simulink model "first_tap_test"  (Simulink 7.2)
settings: Solver=VariableStepDiscrete  StartTime=0.0  StopTime=50  RelTol=1e-3
undefined symbols (not defined in the file or in its folder): pfb_coeff_gen_calc
libraries: xbsIndex_r4 x45, casper_library_misc x3, casper_library_delays x2, simulink x1
settings Model: Creator=User  LastModifiedBy=root
settings OptimizationCC: InitFltsAndDblsToZero=on
settings DebuggingCC: SaveWithDisabledLinksMsg=none  SaveWithParameterizedLinksMsg=none

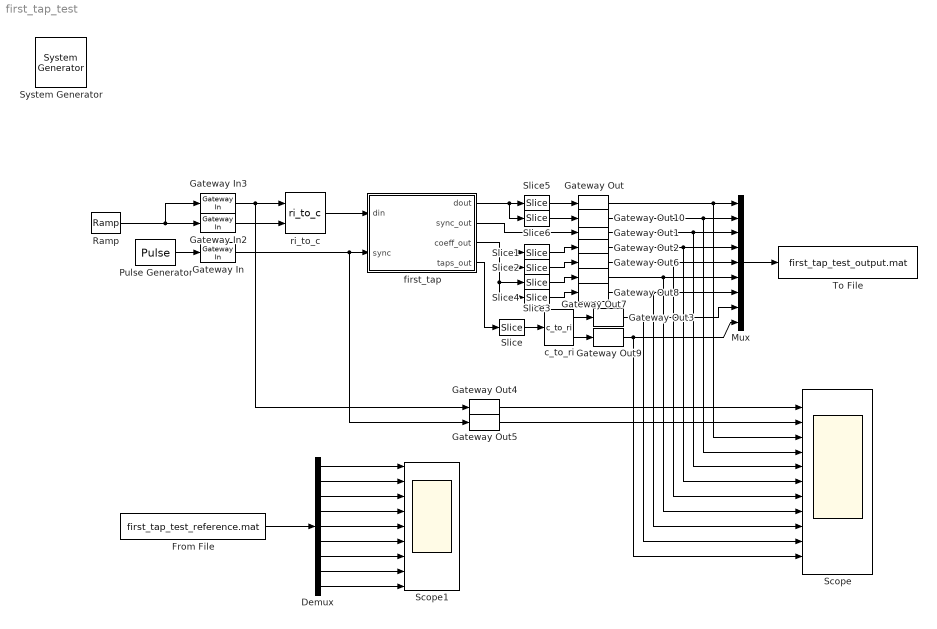
== system first_tap_test ==
  " System Generator" : xbsIndex_r4/ System Generator  Tag=genX  SystemSampleTime=-1  xilinxfamily=Virtex4  part=xc4vsx35  speed=-10  package=ff668  synthesis_tool=XST  clock_wrapper=Clock Enables  directory=./netlist  testbench=off  simulink_period=1  sysclk_period=100  dcm_input_clock_period=100  incr_netlist=off  trim_vbits=Everywhere in SubSystem  dbl_ovrd=According to Block Masks  core_generation=According to Block Masks  run_coregen=off  deprecated_control=off  eval_field=0  block_type=sysgen
      settings: block_version=10.1.1
  Demux : Demux  Outputs=9
  From File : FromFile  FileName=first_tap_test_reference.mat  SampleTime=1
  Gateway In : xbsIndex_r4/Gateway In  arith_type=Boolean  n_bits=16  bin_pt=14  quantization="Round  (unbiased: +/- Inf)"  overflow=Saturate  period=1  dbl_ovrd=off  timing_constraint=None  locs_specified=off  LOCs={}  hdl_port=on  block_type=gatewayin
      settings: infoedit="Gateway in block.  Converts inputs of type Simulink integer, double and fixed point to  Xilinx fixed point type.<P><P>Hardware notes:  In hardware these blocks become top level input ports."  block_version=10.1.1
  Gateway In2 : xbsIndex_r4/Gateway In  arith_type="Signed  (2's comp)"  n_bits=8  bin_pt=7  quantization=Truncate  overflow=Wrap  period=1  dbl_ovrd=off  timing_constraint=None  locs_specified=off  LOCs={}  hdl_port=on  block_type=gatewayin
      settings: infoedit="Gateway in block.  Converts inputs of type Simulink integer, double and fixed point to  Xilinx fixed point type.<P><P>Hardware notes:  In hardware these blocks become top level input ports."  block_version=10.1.1
  Gateway In3 : xbsIndex_r4/Gateway In  arith_type="Signed  (2's comp)"  n_bits=8  bin_pt=7  quantization=Truncate  overflow=Wrap  period=1  dbl_ovrd=off  timing_constraint=None  locs_specified=off  LOCs={}  hdl_port=on  block_type=gatewayin
      settings: infoedit="Gateway in block.  Converts inputs of type Simulink integer, double and fixed point to  Xilinx fixed point type.<P><P>Hardware notes:  In hardware these blocks become top level input ports."  block_version=10.1.1
  Gateway Out{,1..10} (11 alike) : xbsIndex_r4/Gateway Out  hdl_port=on  timing_constraint=None  locs_specified=off  LOCs={}  block_type=gatewayout
      settings: infoedit="Gateway out block.  Converts Xilinx fixed point inputs into ouputs of type Simulink integer, double, or fixed point.<P><P>Hardware notes:  In hardware these blocks become top level output ports or are discarded, depending on how they are configured."  block_version=10.1.1
  Mux : Mux  Inputs=9
  Pulse Generator : DiscretePulseGenerator  Period=16  PhaseDelay=7
  Ramp : simulink/Sources/Ramp  SystemSampleTime=-1  slope=1/64  start=0  X0=0
  Scope : Scope  NumInputPorts=11
      settings: YMin=-1~-1~-1~-5~-5~-5~-5~-5~-5~-5~-5  YMax=1~2~1~5~5~5~5~5~5~5~5
  Scope1 : Scope  NumInputPorts=9
      settings: YMin=-5~-5~-5~-5~-5~-5~-5~-5~-5  YMax=5~5~5~5~5~5~5~5~5
  Slice : xbsIndex_r4/Slice  nbits=28  boolean_output=off  mode=Upper Bit Location + Width  bit1=0  base1=MSB of Input  bit0=0  base0=LSB of Input  dbl_ovrd=off  block_type=slice
      settings: infoedit="Extracts a given range of bits from each input sample and presents it at the output.  The output type is ordinarily unsigned with binary point at zero, but can be Boolean when the slice is one bit wide.<P><P>Hardware notes: In hardware this block costs nothing."  block_version=10.1.1
  Slice1 : xbsIndex_r4/Slice  nbits=6  boolean_output=off  mode=Two Bit Locations  bit1=0  base1=MSB of Input  bit0=-5  base0=MSB of Input  dbl_ovrd=off  block_type=slice
      settings: infoedit="Extracts a given range of bits from each input sample and presents it at the output.  The output type is ordinarily unsigned with binary point at zero, but can be Boolean when the slice is one bit wide.<P><P>Hardware notes: In hardware this block costs nothing."  block_version=10.1.1
  Slice2 : xbsIndex_r4/Slice  nbits=6  boolean_output=off  mode=Two Bit Locations  bit1=-6  base1=MSB of Input  bit0=-11  base0=MSB of Input  dbl_ovrd=off  block_type=slice
      settings: infoedit="Extracts a given range of bits from each input sample and presents it at the output.  The output type is ordinarily unsigned with binary point at zero, but can be Boolean when the slice is one bit wide.<P><P>Hardware notes: In hardware this block costs nothing."  block_version=10.1.1
  Slice3 : xbsIndex_r4/Slice  nbits=6  boolean_output=off  mode=Two Bit Locations  bit1=-12  base1=MSB of Input  bit0=-17  base0=MSB of Input  dbl_ovrd=off  block_type=slice
      settings: infoedit="Extracts a given range of bits from each input sample and presents it at the output.  The output type is ordinarily unsigned with binary point at zero, but can be Boolean when the slice is one bit wide.<P><P>Hardware notes: In hardware this block costs nothing."  block_version=10.1.1
  Slice4 : xbsIndex_r4/Slice  nbits=6  boolean_output=off  mode=Two Bit Locations  bit1=-18  base1=MSB of Input  bit0=-23  base0=MSB of Input  dbl_ovrd=off  block_type=slice
      settings: infoedit="Extracts a given range of bits from each input sample and presents it at the output.  The output type is ordinarily unsigned with binary point at zero, but can be Boolean when the slice is one bit wide.<P><P>Hardware notes: In hardware this block costs nothing."  block_version=10.1.1
  Slice5 : xbsIndex_r4/Slice  nbits=6  boolean_output=off  mode=Two Bit Locations  bit1=0  base1=MSB of Input  bit0=-7  base0=MSB of Input  dbl_ovrd=off  block_type=slice
      settings: infoedit="Extracts a given range of bits from each input sample and presents it at the output.  The output type is ordinarily unsigned with binary point at zero, but can be Boolean when the slice is one bit wide.<P><P>Hardware notes: In hardware this block costs nothing."  block_version=10.1.1
  Slice6 : xbsIndex_r4/Slice  nbits=6  boolean_output=off  mode=Two Bit Locations  bit1=0  base1=MSB of Input  bit0=-7  base0=MSB of Input  dbl_ovrd=off  block_type=slice
      settings: infoedit="Extracts a given range of bits from each input sample and presents it at the output.  The output type is ordinarily unsigned with binary point at zero, but can be Boolean when the slice is one bit wide.<P><P>Hardware notes: In hardware this block costs nothing."  block_version=10.1.1
  To File : ToFile  Filename=first_tap_test_output.mat  MatrixName=output
  c_to_ri : casper_library_misc/c_to_ri  SystemSampleTime=-1  n_bits=14  bin_pt=12
      settings: AttributesFormatString=14_12 r/i
  first_tap : Subsystem  AncestorBlock=casper_library_pfbs/first_tap  mask(first_tap){nput=0, PFBSize=5, CoeffBitWidth=6, TotalTaps=5, BitWidthIn=8, CoeffDistMem=1, WindowType=bartlett, mult_latency=3, bram_latency=2, n_inputs=1, fwidth=1, use_hdl=off, use_embedded=off}
      mask prompts: nput "This is input number:"; PFBSize "Size of PFB: (2^? pnts)"; CoeffBitWidth "Bitwidth of Coefficients:"; TotalTaps "Total Number of Taps:"; BitWidthIn "Input Bitwidth:"; CoeffDistMem "Implement Coeff Gen in Distributed Memory:"; WindowType "Windowing Function:"; mult_latency "Mult Latency"; bram_latency "BRAM Latency"; n_inputs "Number of Simultaneous Inputs: (2^?)"; fwidth "Bit Width (normal=1)"; use_hdl "Use behavioral HDL for multlipliers"; use_embedded "Use embedded multipliers"
      mask init:
      | first_tap_init(gcb,...
      |     'nput', nput,...
      |     'PFBSize', PFBSize,...
      |     'CoeffBitWidth', CoeffBitWidth,...
      |     'TotalTaps', TotalTaps,...
      |     'BitWidthIn', BitWidthIn,...
      |     'CoeffDistMem', CoeffDistMem,...
      |     'WindowType', WindowType,...
      |     'mult_latency', mult_latency,...
      |     'bram_latency', bram_latency,...
      |     'n_inputs', n_inputs,...
      |     'fwidth', fwidth,...
      |     'use_hdl', use_hdl,...
      |     'use_embedded', use_embedded);
      settings: AttributesFormatString=input=0, taps=5
      mask StyleString: edit,edit,edit,edit,edit,edit,popup(bartlett|barthannwin|blackman|blackmanharris|bohamwin|chebwin|flattopwin|gausswin|hamming|hann|kaiser|nuttallwin|parzenwin|rectwin|tukeywin|triang),edit,edit,edit,edit,checkbox,checkbox
      mask CallbackString:
      | |||||||||||use_hdl = get_param(gcb,'use_hdl');
      | if( strcmp(use_hdl,'on')),
      |     set_param(gcb, 'use_embedded','off');
      |     set_param(gcb, 'MaskVisibilities',{'on','on','on','on','on','on','on','on','on','on','on','on','off'});
      | else,
      |     set_param(gcb, 'MaskVisibilities',{'on','on','on','on','on','on','on','on','on','on','on','on','on'});
      | end
      | |
  ri_to_c : casper_library_misc/ri_to_c  SystemSampleTime=-1
  wires:
  Pulse Generator/1 -> Gateway In/1
  Gateway In/1 -> Gateway Out5/1, first_tap/2(sync)
  Ramp/1 -> Gateway In2/1, Gateway In3/1
  c_to_ri/1 -> Gateway Out3/1
  Gateway Out4/1 -> Scope/1
  Gateway Out5/1 -> Scope/2
  Gateway Out/1 -> Scope/3, Mux/1
  Gateway Out3/1 -> Scope/10, Mux/8
  Gateway In3/1 -> Gateway Out4/1, ri_to_c/1
  Gateway In2/1 -> ri_to_c/2
  c_to_ri/2 -> Gateway Out9/1
  Gateway Out9/1 -> Scope/11, Mux/9
  Slice/1 -> c_to_ri/1
  ri_to_c/1 -> first_tap/1(din)
  first_tap/1(dout) -> Slice5/1, Slice6/1
  first_tap/2(sync_out) -> Gateway Out1/1
  first_tap/4(taps_out) -> Slice/1
  first_tap/3(coeff_out) -> Slice1/1, Slice2/1, Slice3/1, Slice4/1
  Slice1/1 -> Gateway Out2/1
  Slice2/1 -> Gateway Out6/1
  Slice3/1 -> Gateway Out7/1
  Slice4/1 -> Gateway Out8/1
  Slice5/1 -> Gateway Out/1
  Slice6/1 -> Gateway Out10/1
  Gateway Out10/1 -> Scope/4, Mux/2
  Gateway Out1/1 -> Scope/5, Mux/3
  Gateway Out2/1 -> Scope/6, Mux/4
  Gateway Out6/1 -> Scope/7, Mux/5
  Gateway Out7/1 -> Scope/8, Mux/6
  Gateway Out8/1 -> Scope/9, Mux/7
  Mux/1 -> To File/1
  From File/1 -> Demux/1
  Demux/1 -> Scope1/1
  Demux/2 -> Scope1/2
  Demux/3 -> Scope1/3
  Demux/4 -> Scope1/4
  Demux/5 -> Scope1/5
  Demux/6 -> Scope1/6
  Demux/7 -> Scope1/7
  Demux/8 -> Scope1/8
  Demux/9 -> Scope1/9

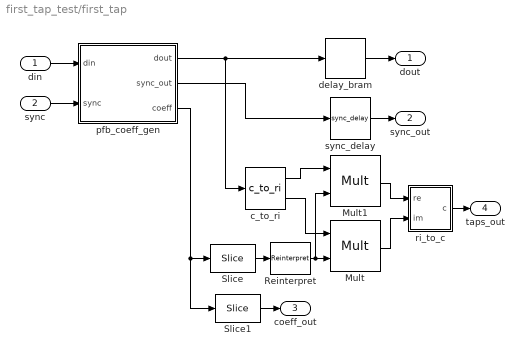
== system first_tap_test/first_tap ==
  din : Inport  OutDataType=sfix(16)  OutScaling=2^0
  sync : Inport  Port=2  OutDataType=sfix(16)  OutScaling=2^0
  Mult : xbsIndex_r4/Mult  precision=Full  arith_type="Signed  (2's comp)"  n_bits=8  bin_pt=2  quantization=Truncate  overflow=Wrap  en=off  latency=mult_latency  dbl_ovrd=off  use_behavioral_HDL=off  opt=Speed  use_embedded=off  optimum_pipeline=off  pipeline=on  use_rpm=on  placement_style=Rectangular shape  block_type=mult
      settings: infoedit=Hardware notes: To use the internal pipeline stage of the dedicated multiplier you must select 'Pipeline for maximum performance'.  xl_area=[0, 0, 0, 0, 0, 0, 0]  block_version=9.1.01
  Mult1 : xbsIndex_r4/Mult  precision=Full  arith_type="Signed  (2's comp)"  n_bits=8  bin_pt=2  quantization=Truncate  overflow=Wrap  en=off  latency=mult_latency  dbl_ovrd=off  use_behavioral_HDL=off  opt=Speed  use_embedded=off  optimum_pipeline=off  pipeline=on  use_rpm=on  placement_style=Rectangular shape  block_type=mult
      settings: infoedit=Hardware notes: To use the internal pipeline stage of the dedicated multiplier you must select 'Pipeline for maximum performance'.  xl_area=[0, 0, 0, 0, 0, 0, 0]  block_version=9.1.01
  Reinterpret : xbsIndex_r4/Reinterpret  force_arith_type=on  arith_type="Signed  (2's comp)"  force_bin_pt=on  bin_pt=CoeffBitWidth - 1  block_type=reinterpret
      settings: infoedit="Changes signal type without altering the binary representation.   You can changed the signal between signed and unsigned, and relocate the binary point.<P><P>Hardware notes: In hardware this block costs nothing.<P><P>Example:  Suppose the input is 6 bits wide, signed, with 2 fractional bits, and the output is forced to unsigned with 0 fractional bits.  Then an input of -2.0 (1110.00 in binary 2's complement) becomes an output of 56 (111000 in binary)."  block_version=9.1.01
  Slice : xbsIndex_r4/Slice  nbits=CoeffBitWidth  boolean_output=off  mode=Lower Bit Location + Width  bit1=0  base1=MSB of Input  bit0=0  base0=LSB of Input  dbl_ovrd=off  block_type=slice
      settings: infoedit="Extracts a given range of bits from each input sample and presents it at the output.  The output type is ordinarily unsigned with binary point at zero, but can be Boolean when the slice is one bit wide.<P><P>Hardware notes: In hardware this block costs nothing."  block_version=9.1.01
  Slice1 : xbsIndex_r4/Slice  nbits=CoeffBitWidth * (TotalTaps - 1)  boolean_output=off  mode=Two Bit Locations  bit1=0  base1=MSB of Input  bit0=CoeffBitWidth  base0=LSB of Input  dbl_ovrd=off  block_type=slice
      settings: infoedit="Extracts a given range of bits from each input sample and presents it at the output.  The output type is ordinarily unsigned with binary point at zero, but can be Boolean when the slice is one bit wide.<P><P>Hardware notes: In hardware this block costs nothing."  block_version=9.1.01
  c_to_ri : casper_library_misc/c_to_ri  SystemSampleTime=-1  n_bits=BitWidthIn  bin_pt=BitWidthIn-1
      settings: AttributesFormatString=8_7 r/i
  delay_bram : casper_library_delays/delay_bram  SystemSampleTime=-1  DelayLen=2^(PFBSize-n_inputs)  bram_latency=bram_latency
  pfb_coeff_gen : Subsystem  AncestorBlock=casper_library_pfbs/pfb_coeff_gen  mask(pfb_coeff_gen){PFBSize=5, CoeffBitWidth=6, TotalTaps=5, CoeffDistMem=1, WindowType=bartlett, bram_latency=2, n_inputs=1, nput=0, fwidth=1}
      mask prompts: PFBSize "Size of PFB: (2^? pnts)"; CoeffBitWidth "Bitwidth of Coefficients:"; TotalTaps "Total Number of Taps:"; CoeffDistMem "Implement Coeff Gen in Distributed Memory"; WindowType "Windowing Function:"; bram_latency "BRAM Latency"; n_inputs "Number of Simultaneous Inputs: (2^?)"; nput "This is input number:"; fwidth "Bin Width (normal=1)"
      mask init:
      | pfb_coeff_gen_init(gcb, ...
      |     'PFBSize', PFBSize, ...
      |     'CoeffBitWidth', CoeffBitWidth, ...
      |     'TotalTaps', TotalTaps, ...
      |     'CoeffDistMem', CoeffDistMem, ...
      |     'WindowType', WindowType, ...
      |     'bram_latency', bram_latency, ...
      |     'n_inputs', n_inputs, ...
      |     'nput', nput, ...
      |     'fwidth', fwidth);
      settings: AttributesFormatString=PFBSize=5, n_inputs=1, taps=5
  ri_to_c : Subsystem
  sync_delay : casper_library_delays/sync_delay  SystemSampleTime=-1  DelayLen=2^(PFBSize-n_inputs)
  dout : Outport  OutDataType=sfix(16)  OutScaling=2^0
  sync_out : Outport  Port=2  OutDataType=sfix(16)  OutScaling=2^0
  coeff_out : Outport  Port=3  OutDataType=sfix(16)  OutScaling=2^0
  taps_out : Outport  Port=4  OutDataType=sfix(16)  OutScaling=2^0
  wires:
  ri_to_c/1(c) -> taps_out/1
  Mult/1 -> ri_to_c/2(im)
  Mult1/1 -> ri_to_c/1(re)
  c_to_ri/2 -> Mult/1
  c_to_ri/1 -> Mult1/1
  pfb_coeff_gen/3(coeff) -> Slice1/1, Slice/1
  pfb_coeff_gen/2(sync_out) -> sync_delay/1
  sync/1 -> pfb_coeff_gen/2(sync)
  pfb_coeff_gen/1(dout) -> delay_bram/1, c_to_ri/1
  din/1 -> pfb_coeff_gen/1(din)
  delay_bram/1 -> dout/1
  sync_delay/1 -> sync_out/1
  Slice1/1 -> coeff_out/1
  Slice/1 -> Reinterpret/1
  Reinterpret/1 -> Mult1/2, Mult/2

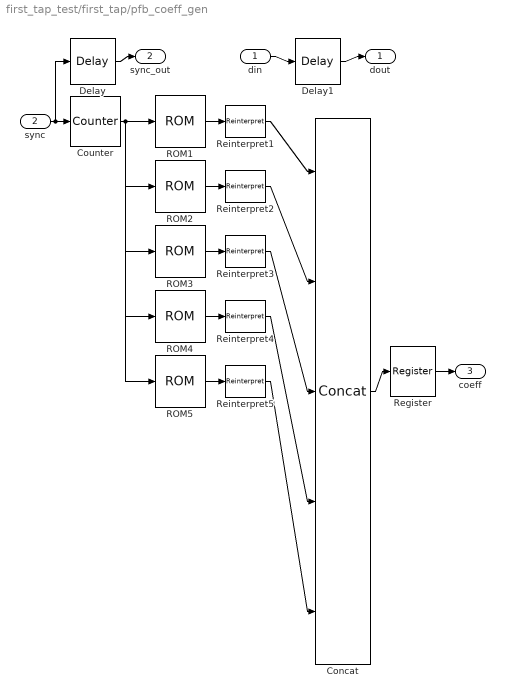
== system first_tap_test/first_tap/pfb_coeff_gen ==
  din : Inport  OutDataType=sfix(16)  OutScaling=2^0
  sync : Inport  Port=2  OutDataType=sfix(16)  OutScaling=2^0
  Concat : xbsIndex_r4/Concat  num_inputs=5  dbl_ovrd=off  block_type=concat
      settings: block_version=9.1.01
  Counter : xbsIndex_r4/Counter  cnt_type=Free Running  cnt_to=Inf  operation=Up  start_count=0  cnt_by_val=1  arith_type=Unsigned  n_bits=4  bin_pt=0  load_pin=off  rst=on  en=off  explicit_period=on  period=1  dbl_ovrd=off  use_behavioral_HDL=off  implementation=Fabric  use_rpm=on  block_type=counter
      settings: xl_area=[0, 0, 0, 0, 0, 0, 0]  block_version=9.1.01
  Delay : xbsIndex_r4/Delay  en=off  latency=bram_latency+1  dbl_ovrd=off  reg_retiming=off  block_type=delay
      settings: xl_area=[0, 0, 0, 0, 0, 0, 0]  block_version=9.1.01
  Delay1 : xbsIndex_r4/Delay  en=off  latency=3  dbl_ovrd=off  reg_retiming=off  block_type=delay
      settings: xl_area=[0, 0, 0, 0, 0, 0, 0]  block_version=9.1.01
  ROM1 : xbsIndex_r4/ROM  depth=16  initVector=pfb_coeff_gen_calc(5, 5,'bartlett',1, 0,1,1)  distributed_mem=Distributed memory  rst=off  init_reg=0  en=off  latency=2  arith_type="Signed  (2's comp)"  n_bits=6  bin_pt=5  dbl_ovrd=off  optimize=Area  use_rpm=on  block_type=sprom
      settings: xl_area=[0, 0, 0, 0, 0, 0, 0]
  ROM2 : xbsIndex_r4/ROM  depth=16  initVector=pfb_coeff_gen_calc(5, 5,'bartlett',1, 0,1,2)  distributed_mem=Distributed memory  rst=off  init_reg=0  en=off  latency=2  arith_type="Signed  (2's comp)"  n_bits=6  bin_pt=5  dbl_ovrd=off  optimize=Area  use_rpm=on  block_type=sprom
      settings: xl_area=[0, 0, 0, 0, 0, 0, 0]
  ROM3 : xbsIndex_r4/ROM  depth=16  initVector=pfb_coeff_gen_calc(5, 5,'bartlett',1, 0,1,3)  distributed_mem=Distributed memory  rst=off  init_reg=0  en=off  latency=2  arith_type="Signed  (2's comp)"  n_bits=6  bin_pt=5  dbl_ovrd=off  optimize=Area  use_rpm=on  block_type=sprom
      settings: xl_area=[0, 0, 0, 0, 0, 0, 0]
  ROM4 : xbsIndex_r4/ROM  depth=16  initVector=pfb_coeff_gen_calc(5, 5,'bartlett',1, 0,1,4)  distributed_mem=Distributed memory  rst=off  init_reg=0  en=off  latency=2  arith_type="Signed  (2's comp)"  n_bits=6  bin_pt=5  dbl_ovrd=off  optimize=Area  use_rpm=on  block_type=sprom
      settings: xl_area=[0, 0, 0, 0, 0, 0, 0]
  ROM5 : xbsIndex_r4/ROM  depth=16  initVector=pfb_coeff_gen_calc(5, 5,'bartlett',1, 0,1,5)  distributed_mem=Distributed memory  rst=off  init_reg=0  en=off  latency=2  arith_type="Signed  (2's comp)"  n_bits=6  bin_pt=5  dbl_ovrd=off  optimize=Area  use_rpm=on  block_type=sprom
      settings: block_version=11.4
  Register : xbsIndex_r4/Register  init=0  rst=off  en=off  dbl_ovrd=off  block_type=register
      settings: xl_area=[0, 0, 0, 0, 0, 0, 0]  block_version=9.1.01
  Reinterpret{1..5} (5 alike) : xbsIndex_r4/Reinterpret  force_arith_type=on  arith_type=Unsigned  force_bin_pt=on  bin_pt=0  block_type=reinterpret
      Reinterpret1 settings: infoedit="Changes signal type without altering the binary representation.   You can changed the signal between signed and unsigned, and relocate the binary point.<P><P>Hardware notes: In hardware this block costs nothing.<P><P>Example:  Suppose the input is 6 bits wide, signed, with 2 fractional bits, and the output is forced to unsigned with 0 fractional bits.  Then an input of -2.0 (1110.00 in binary 2's complement) becomes an output of 56 (111000 in binary)."  block_version=9.1.01
      Reinterpret2 settings: infoedit="Changes signal type without altering the binary representation.   You can changed the signal between signed and unsigned, and relocate the binary point.<P><P>Hardware notes: In hardware this block costs nothing.<P><P>Example:  Suppose the input is 6 bits wide, signed, with 2 fractional bits, and the output is forced to unsigned with 0 fractional bits.  Then an input of -2.0 (1110.00 in binary 2's complement) becomes an output of 56 (111000 in binary)."  block_version=9.1.01
      Reinterpret3 settings: infoedit="Changes signal type without altering the binary representation.   You can changed the signal between signed and unsigned, and relocate the binary point.<P><P>Hardware notes: In hardware this block costs nothing.<P><P>Example:  Suppose the input is 6 bits wide, signed, with 2 fractional bits, and the output is forced to unsigned with 0 fractional bits.  Then an input of -2.0 (1110.00 in binary 2's complement) becomes an output of 56 (111000 in binary)."  block_version=9.1.01
      Reinterpret4 settings: infoedit="Changes signal type without altering the binary representation.   You can changed the signal between signed and unsigned, and relocate the binary point.<P><P>Hardware notes: In hardware this block costs nothing.<P><P>Example:  Suppose the input is 6 bits wide, signed, with 2 fractional bits, and the output is forced to unsigned with 0 fractional bits.  Then an input of -2.0 (1110.00 in binary 2's complement) becomes an output of 56 (111000 in binary)."  block_version=9.1.01
      Reinterpret5 settings: infoedit="Changes signal type without altering the binary representation.   You can changed the signal between signed and unsigned, and relocate the binary point.<br><br>Hardware notes: In hardware this block costs nothing.<br><br>Example:  Suppose the input is 6 bits wide, signed, with 2 fractional bits, and the output is forced to unsigned with 0 fractional bits.  Then an input of -2.0 (1110.00 in binary 2's complement) becomes an output of 56 (111000 in binary)."
  dout : Outport  OutDataType=sfix(16)  OutScaling=2^0
  sync_out : Outport  Port=2  OutDataType=sfix(16)  OutScaling=2^0
  coeff : Outport  Port=3  OutDataType=sfix(16)  OutScaling=2^0
  wires:
  din/1 -> Delay1/1
  Delay1/1 -> dout/1
  sync/1 -> Counter/1, Delay/1
  Delay/1 -> sync_out/1
  Concat/1 -> Register/1
  Register/1 -> coeff/1
  Counter/1 -> ROM1/1, ROM2/1, ROM3/1, ROM4/1, ROM5/1
  ROM1/1 -> Reinterpret1/1
  Reinterpret1/1 -> Concat/1
  ROM2/1 -> Reinterpret2/1
  Reinterpret2/1 -> Concat/2
  ROM3/1 -> Reinterpret3/1
  Reinterpret3/1 -> Concat/3
  ROM4/1 -> Reinterpret4/1
  Reinterpret4/1 -> Concat/4
  ROM5/1 -> Reinterpret5/1
  Reinterpret5/1 -> Concat/5

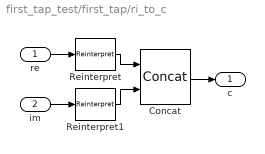
== system first_tap_test/first_tap/ri_to_c ==
  re : Inport  OutDataType=sfix(16)  OutScaling=2^0
  im : Inport  Port=2  OutDataType=sfix(16)  OutScaling=2^0
  Concat : xbsIndex_r4/Concat  num_inputs=2  dbl_ovrd=off  block_type=concat
      settings: block_version=9.1.01
  Reinterpret : xbsIndex_r4/Reinterpret  force_arith_type=on  arith_type=Unsigned  force_bin_pt=on  bin_pt=0  block_type=reinterpret
      settings: infoedit="Changes signal type without altering the binary representation.   You can changed the signal between signed and unsigned, and relocate the binary point.<P><P>Hardware notes: In hardware this block costs nothing.<P><P>Example:  Suppose the input is 6 bits wide, signed, with 2 fractional bits, and the output is forced to unsigned with 0 fractional bits.  Then an input of -2.0 (1110.00 in binary 2's complement) becomes an output of 56 (111000 in binary)."  block_version=9.1.01
  Reinterpret1 : xbsIndex_r4/Reinterpret  force_arith_type=on  arith_type=Unsigned  force_bin_pt=on  bin_pt=0  block_type=reinterpret
      settings: infoedit="Changes signal type without altering the binary representation.   You can changed the signal between signed and unsigned, and relocate the binary point.<P><P>Hardware notes: In hardware this block costs nothing.<P><P>Example:  Suppose the input is 6 bits wide, signed, with 2 fractional bits, and the output is forced to unsigned with 0 fractional bits.  Then an input of -2.0 (1110.00 in binary 2's complement) becomes an output of 56 (111000 in binary)."  block_version=9.1.01
  c : Outport  OutDataType=sfix(16)  OutScaling=2^0
  wires:
  Reinterpret/1 -> Concat/1
  Reinterpret1/1 -> Concat/2
  re/1 -> Reinterpret/1
  Concat/1 -> c/1
  im/1 -> Reinterpret1/1
